simulink model "Stufe5_Laengsdyn3DOF"  (R2026b)
settings: Solver=ode45  StopTime=4.5  MaxStep=0.01  RelTol=1e-6
undefined symbols (not defined in the file or in its folder): PAR_Ach_AbstHi_f64, PAR_Ach_AbstVo_f64, PAR_Ach_BeschlBrems_f64, PAR_Ach_SchwerpHoehe_f64, PAR_Ach_ZeitBrems_f64, PAR_Auf_DaempfHi_f64, PAR_Auf_DaempfVo_f64, PAR_Auf_FederHi_f64, PAR_Auf_FederVo_f64, PAR_Auf_TraeghNick_f64, PAR_Lng_BeschlErde_f64, PAR_Lng_GeschwStart_f64, PAR_Lng_MasseFzg_f64
libraries: simulink x1

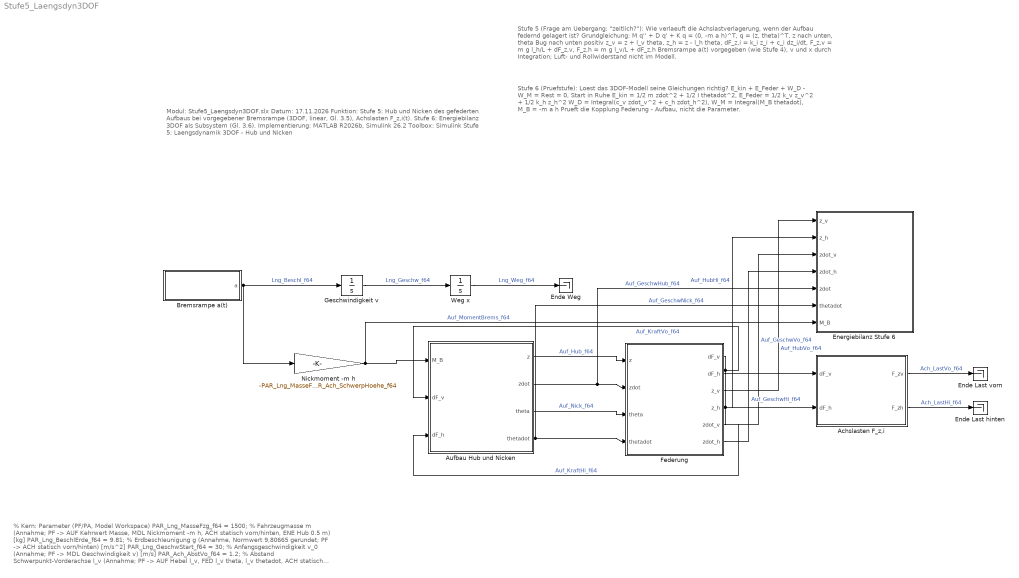
== system Stufe5_Laengsdyn3DOF ==
  note: % Kern: Parameter (PF/PA, Model Workspace)
      | PAR_Lng_MasseFzg_f64 = 1500; % Fahrzeugmasse m (Annahme; PF -> AUF Kehrwert Masse, MDL Nickmoment -m h, ACH statisch vorn/hinten, ENE Hub 0.5 m) [kg]
      | PAR_Lng_BeschlErde_f64 = 9.81; % Erdbeschleunigung g (Annahme, Normwert 9,80665 gerundet; PF -> ACH statisch vorn/hinten) [m/s^2]
      | PAR_Lng_GeschwStart_f64 = 30; % Anfangsgeschwindigkeit v_0 (Annahme; PF -> MDL Geschwindigkeit v) [m/s]
      | PAR_Ach_AbstVo_f64 = 1.2; % Abstand Schwerpunkt-Vorderachse l_v (Annahme; PF -> AUF Hebel l_v, FED l_v theta, l_v thetadot, ACH statisch vorn/hinten) [m]
      | PAR_Ach_AbstHi_f64 = 1.5; % Abstand Schwerpunkt-Hinterachse l_h (Annahme; PF -> AUF Hebel l_h, FED l_h theta, l_h thetadot, ACH statisch vorn/hinten) [m]
      | PAR_Ach_SchwerpHoehe_f64 = 0.55; % Schwerpunkthoehe h (Lit [MW14, Abb. 8.5], Interpretation; PF -> MDL Nickmoment -m h) [m]
      | PAR_Ach_BeschlBrems_f64 = 8; % Betrag der Bremsverzoegerung a_B (Annahme; PA -> BR Rampe, Begrenzung -a_B) [m/s^2]
      | PAR_Ach_ZeitBrems_f64 = 0.3; % Aufbauzeit der Bremsverzoegerung t_r (Annahme; PA -> BR Rampe) [s]
      | PAR_Ach_ZeitStart_f64 = 1; % Beginn der Bremsrampe (Annahme; PA -> BR Rampe) [s]
      | PAR_Auf_FederVo_f64 = 50000; % Federkonstante Vorderachse k_v, beide Raeder (Annahme; PA -> FED Feder k_v, ENE Feder 0.5 k_v) [N/m]
      | PAR_Auf_FederHi_f64 = 45000; % Federkonstante Hinterachse k_h, beide Raeder (Annahme; PA -> FED Feder k_h, ENE Feder 0.5 k_h) [N/m]
      | PAR_Auf_DaempfVo_f64 = 4000; % Daempferkonstante Vorderachse c_v, beide Raeder (Annahme; PA -> FED Daempfer c_v, ENE Daempfer c_v) [N s/m]
      | PAR_Auf_DaempfHi_f64 = 4000; % Daempferkonstante Hinterachse c_h, beide Raeder (Annahme; PA -> FED Daempfer c_h, ENE Daempfer c_h) [N s/m]
      | PAR_Auf_TraeghNick_f64 = 2500; % Nicktraegheitsmoment I um die Querachse (Annahme; PA -> AUF Kehrwert I, ENE Nicken 0.5 I) [kg m^2]
      | % Kern: Signale Stufe 5 (MDL)
      | Lng_Beschl_f64 = '0 -> -8' ; % Beschleunigung a, Bremsrampe, geloggt (MDL; Bremsrampe a(t):1 -> Geschwindigkeit v:1, Nickmoment -m h:1) [m/s^2]
      | Lng_Geschw_f64 = '30 -> 3.2' ; % Geschwindigkeit v, geloggt (MDL; Geschwindigkeit v:1 -> Weg x:1) [m/s]
      | Lng_Weg_f64 = '0 -> 90.08' ; % Weg x, geloggt (MDL; Weg x:1 -> Ende Weg:1) [m]
      | Auf_MomentBrems_f64 = '0 -> 6600' ; % Nickmoment -m a h, geloggt (MDL; Nickmoment -m h:1 -> Aufbau Hub und Nicken:1, Energiebilanz Stufe 6:7) [N m]
      | Auf_Hub_f64 = '0 -> 0.0030 (max 0.0054)' ; % Hub z, nach unten positiv, geloggt (MDL; Aufbau Hub und Nicken:1 -> Federung:1) [m]
      | Auf_GeschwHub_f64 = '0 -> 0 (max 0.0177)' ; % Hubgeschwindigkeit zdot, geloggt (MDL; Aufbau Hub und Nicken:2 -> Federung:2, Energiebilanz Stufe 6:5) [m/s]
      | Auf_Nick_f64 = '0 -> 0.0382 (max 0.0473)' ; % Nickwinkel theta, Bug nach unten positiv, geloggt (MDL; Aufbau Hub und Nicken:3 -> Federung:3) [rad]
      | Auf_GeschwNick_f64 = '0 -> 0 (max 0.154)' ; % Nickgeschwindigkeit thetadot, geloggt (MDL; Aufbau Hub und Nicken:4 -> Federung:4, Energiebilanz Stufe 6:6) [rad/s]
      | Auf_KraftVo_f64 = '0 -> 2444 (max 3261)' ; % Federungskraft vorn dF_z,v = k_v z_v + c_v zdot_v (MDL; Federung:1 -> Aufbau Hub und Nicken:2, Achslasten F_z,i:1) [N]
      | Auf_KraftHi_f64 = '0 -> -2444 (min -3147)' ; % Federungskraft hinten dF_z,h = k_h z_h + c_h zdot_h (MDL; Federung:2 -> Aufbau Hub und Nicken:3, Achslasten F_z,i:2) [N]
      | Ach_LastVo_f64 = '8175 -> 10619 (max 11436)' ; % Achslast vorn F_z,v = m g l_h/L + dF_z,v, geloggt (MDL; Achslasten F_z,i:1 -> Ende Last vorn:1) [N]
      | Ach_LastHi_f64 = '6540 -> 4095 (min 3393)' ; % Achslast hinten F_z,h = m g l_v/L + dF_z,h, geloggt (MDL; Achslasten F_z,i:2 -> Ende Last hinten:1) [N]
  note: Modul: Stufe5_Laengsdyn3DOF.slx
      | Datum: 17.11.2026
      | Funktion: Stufe 5: Hub und Nicken des gefederten Aufbaus bei vorgegebener
      | Bremsrampe (3DOF, linear, Gl. 3.5), Achslasten F_z,i(t).
      | Stufe 6: Energiebilanz 3DOF als Subsystem (Gl. 3.6).
      | Implementierung: MATLAB R2026b, Simulink 26.2
      | Toolbox: Simulink
      |
      | Stufe 5: Laengsdynamik 3DOF - Hub und Nicken
  note: Stufe 5 (Frage am Uebergang: "zeitlich?"): Wie verlaeuft die Achslastverlagerung, wenn der Aufbau federnd gelagert ist?
      | Grundgleichung: M q'' + D q' + K q = (0, -m a h)^T, q = (z, theta)^T, z nach unten, theta Bug nach unten positiv
      | z_v = z + l_v theta, z_h = z - l_h theta, dF_z,i = k_i z_i + c_i dz_i/dt, F_z,v = m g l_h/L + dF_z,v, F_z,h = m g l_v/L + dF_z,h
      | Bremsrampe a(t) vorgegeben (wie Stufe 4), v und x durch Integration; Luft- und Rollwiderstand nicht im Modell.
  note: Stufe 6 (Pruefstufe): Loest das 3DOF-Modell seine Gleichungen richtig?
      | E_kin + E_Feder + W_D - W_M = Rest = 0, Start in Ruhe
      | E_kin = 1/2 m zdot^2 + 1/2 I thetadot^2, E_Feder = 1/2 k_v z_v^2 + 1/2 k_h z_h^2
      | W_D = Integral(c_v zdot_v^2 + c_h zdot_h^2), W_M = Integral(M_B thetadot), M_B = -m a h
      | Prueft die Kopplung Federung - Aufbau, nicht die Parameter.
  Achslasten F_z,i : Subsystem
  Aufbau Hub und Nicken : Subsystem
  Bremsrampe a(t) : Subsystem
  Ende Last hinten : Terminator
  Ende Last vorn : Terminator
  Ende Weg : Terminator
  Energiebilanz Stufe 6 : Subsystem
  Federung : Subsystem
  Geschwindigkeit v : Integrator  InitialCondition=PAR_Lng_GeschwStart_f64
  Nickmoment -m h : Gain  Gain=-PAR_Lng_MasseFzg_f64*PAR_Ach_SchwerpHoehe_f64
  Weg x : Integrator
  wires:
  Bremsrampe a(t)/1(a) -> Geschwindigkeit v/1, Nickmoment -m h/1  "Lng_Beschl_f64"
  Geschwindigkeit v/1 -> Weg x/1  "Lng_Geschw_f64"
  Weg x/1 -> Ende Weg/1  "Lng_Weg_f64"
  Nickmoment -m h/1 -> Aufbau Hub und Nicken/1(M_B), Energiebilanz Stufe 6/7(M_B)  "Auf_MomentBrems_f64"
  Aufbau Hub und Nicken/1(z) -> Federung/1(z)  "Auf_Hub_f64"
  Aufbau Hub und Nicken/2(zdot) -> Federung/2(zdot), Energiebilanz Stufe 6/5(zdot)  "Auf_GeschwHub_f64"
  Aufbau Hub und Nicken/3(theta) -> Federung/3(theta)  "Auf_Nick_f64"
  Aufbau Hub und Nicken/4(thetadot) -> Federung/4(thetadot), Energiebilanz Stufe 6/6(thetadot)  "Auf_GeschwNick_f64"
  Federung/1(dF_v) -> Aufbau Hub und Nicken/2(dF_v), Achslasten F_z,i/1(dF_v)  "Auf_KraftVo_f64"
  Federung/2(dF_h) -> Aufbau Hub und Nicken/3(dF_h), Achslasten F_z,i/2(dF_h)  "Auf_KraftHi_f64"
  Achslasten F_z,i/1(F_zv) -> Ende Last vorn/1  "Ach_LastVo_f64"
  Achslasten F_z,i/2(F_zh) -> Ende Last hinten/1  "Ach_LastHi_f64"
  Federung/3(z_v) -> Energiebilanz Stufe 6/1(z_v)  "Auf_HubVo_f64"
  Federung/4(z_h) -> Energiebilanz Stufe 6/2(z_h)  "Auf_HubHi_f64"
  Federung/5(zdot_v) -> Energiebilanz Stufe 6/3(zdot_v)  "Auf_GeschwVo_f64"
  Federung/6(zdot_h) -> Energiebilanz Stufe 6/4(zdot_h)  "Auf_GeschwHi_f64"

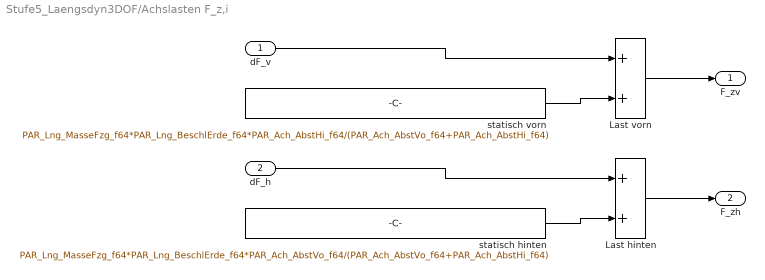
== system Stufe5_Laengsdyn3DOF/Achslasten F_z,i ==
  dF_v : Inport
  dF_h : Inport  Port=2
  Last hinten : Sum
  Last vorn : Sum
  statisch hinten : Constant  Value=PAR_Lng_MasseFzg_f64*PAR_Lng_BeschlErde_f64*PAR_Ach_AbstVo_f64/(PAR_Ach_AbstVo_f64+PAR_Ach_AbstHi_f64)
  statisch vorn : Constant  Value=PAR_Lng_MasseFzg_f64*PAR_Lng_BeschlErde_f64*PAR_Ach_AbstHi_f64/(PAR_Ach_AbstVo_f64+PAR_Ach_AbstHi_f64)
  F_zv : Outport
  F_zh : Outport  Port=2
  wires:
  dF_v/1 -> Last vorn/1
  statisch vorn/1 -> Last vorn/2
  dF_h/1 -> Last hinten/1
  statisch hinten/1 -> Last hinten/2
  Last vorn/1 -> F_zv/1
  Last hinten/1 -> F_zh/1

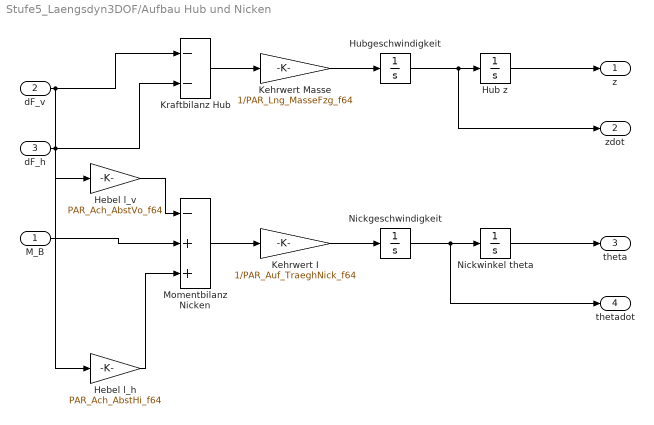
== system Stufe5_Laengsdyn3DOF/Aufbau Hub und Nicken ==
  M_B : Inport
  dF_v : Inport  Port=2
  dF_h : Inport  Port=3
  Hebel l_h : Gain  Gain=PAR_Ach_AbstHi_f64
  Hebel l_v : Gain  Gain=PAR_Ach_AbstVo_f64
  Hub z : Integrator
  Hubgeschwindigkeit : Integrator
  Kehrwert I : Gain  Gain=1/PAR_Auf_TraeghNick_f64
  Kehrwert Masse : Gain  Gain=1/PAR_Lng_MasseFzg_f64
  Kraftbilanz Hub : Sum  Inputs=|--
  Momentbilanz Nicken : Sum  Inputs=-++
  Nickgeschwindigkeit : Integrator
  Nickwinkel theta : Integrator
  z : Outport
  zdot : Outport  Port=2
  theta : Outport  Port=3
  thetadot : Outport  Port=4
  wires:
  dF_v/1 -> Kraftbilanz Hub/1, Hebel l_v/1
  dF_h/1 -> Kraftbilanz Hub/2, Hebel l_h/1
  Kraftbilanz Hub/1 -> Kehrwert Masse/1
  Kehrwert Masse/1 -> Hubgeschwindigkeit/1
  Hubgeschwindigkeit/1 -> Hub z/1, zdot/1
  Hub z/1 -> z/1
  Hebel l_v/1 -> Momentbilanz Nicken/1
  M_B/1 -> Momentbilanz Nicken/2
  Hebel l_h/1 -> Momentbilanz Nicken/3
  Momentbilanz Nicken/1 -> Kehrwert I/1
  Kehrwert I/1 -> Nickgeschwindigkeit/1
  Nickgeschwindigkeit/1 -> Nickwinkel theta/1, thetadot/1
  Nickwinkel theta/1 -> theta/1

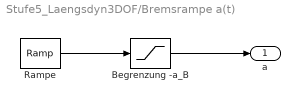
== system Stufe5_Laengsdyn3DOF/Bremsrampe a(t) ==
  Begrenzung -a_B : Saturate  UpperLimit=0  LowerLimit=-PAR_Ach_BeschlBrems_f64
  Rampe : simulink/Sources/Ramp  slope=-PAR_Ach_BeschlBrems_f64/PAR_Ach_ZeitBrems_f64  start=PAR_Ach_ZeitStart_f64  InitialOutput=0
  a : Outport
  wires:
  Rampe/1 -> Begrenzung -a_B/1
  Begrenzung -a_B/1 -> a/1

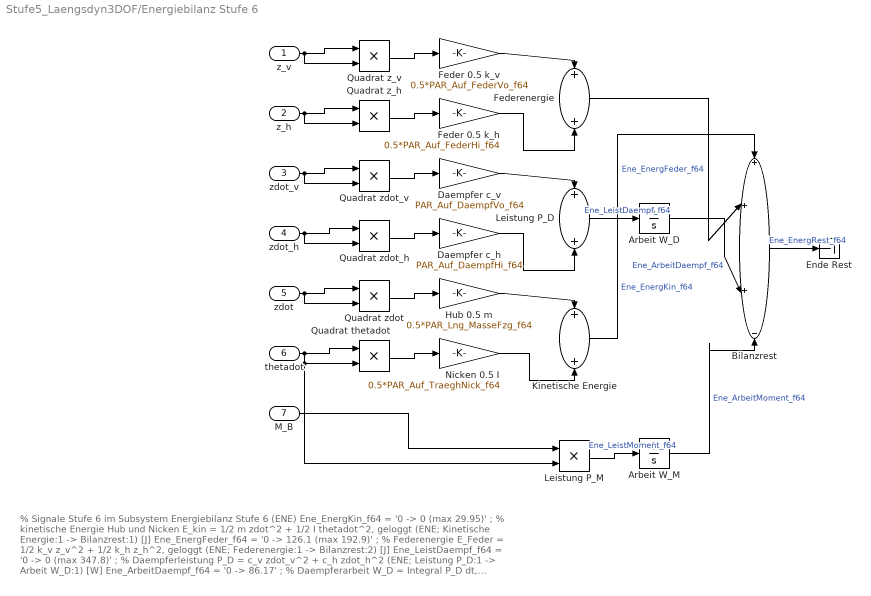
== system Stufe5_Laengsdyn3DOF/Energiebilanz Stufe 6 ==
  note: % Signale Stufe 6 im Subsystem Energiebilanz Stufe 6 (ENE)
      | Ene_EnergKin_f64 = '0 -> 0 (max 29.95)' ; % kinetische Energie Hub und Nicken E_kin = 1/2 m zdot^2 + 1/2 I thetadot^2, geloggt (ENE; Kinetische Energie:1 -> Bilanzrest:1) [J]
      | Ene_EnergFeder_f64 = '0 -> 126.1 (max 192.9)' ; % Federenergie E_Feder = 1/2 k_v z_v^2 + 1/2 k_h z_h^2, geloggt (ENE; Federenergie:1 -> Bilanzrest:2) [J]
      | Ene_LeistDaempf_f64 = '0 -> 0 (max 347.8)' ; % Daempferleistung P_D = c_v zdot_v^2 + c_h zdot_h^2 (ENE; Leistung P_D:1 -> Arbeit W_D:1) [W]
      | Ene_ArbeitDaempf_f64 = '0 -> 86.17' ; % Daempferarbeit W_D = Integral P_D dt, geloggt (ENE; Arbeit W_D:1 -> Bilanzrest:3) [J]
      | Ene_LeistMoment_f64 = '0 -> 0 (max 1019, min -312)' ; % Leistung des Nickmoments P_M = M_B thetadot (ENE; Leistung P_M:1 -> Arbeit W_M:1) [W]
      | Ene_ArbeitMoment_f64 = '0 -> 212.3 (max 271.9)' ; % Arbeit des Nickmoments W_M = Integral P_M dt, geloggt (ENE; Arbeit W_M:1 -> Bilanzrest:4) [J]
      | Ene_EnergRest_f64 = '0 -> -2.9e-07' ; % Bilanzrest E_kin + E_Feder + W_D - W_M, geloggt, Toleranz 3.9e-04 J (ENE; Bilanzrest:1 -> Ende Rest:1) [J]
  z_v : Inport
  z_h : Inport  Port=2
  zdot_v : Inport  Port=3
  zdot_h : Inport  Port=4
  zdot : Inport  Port=5
  thetadot : Inport  Port=6
  M_B : Inport  Port=7
  Arbeit W_D : Integrator
  Arbeit W_M : Integrator
  Bilanzrest : Sum  Inputs=+++-
  Daempfer c_h : Gain  Gain=PAR_Auf_DaempfHi_f64
  Daempfer c_v : Gain  Gain=PAR_Auf_DaempfVo_f64
  Ende Rest : Terminator
  Feder 0.5 k_h : Gain  Gain=0.5*PAR_Auf_FederHi_f64
  Feder 0.5 k_v : Gain  Gain=0.5*PAR_Auf_FederVo_f64
  Federenergie : Sum
  Hub 0.5 m : Gain  Gain=0.5*PAR_Lng_MasseFzg_f64
  Kinetische Energie : Sum
  Leistung P_D : Sum
  Leistung P_M : Product
  Nicken 0.5 I : Gain  Gain=0.5*PAR_Auf_TraeghNick_f64
  Quadrat thetadot : Product
  Quadrat z_h : Product
  Quadrat z_v : Product
  Quadrat zdot : Product
  Quadrat zdot_h : Product
  Quadrat zdot_v : Product
  wires:
  z_v/1 -> Quadrat z_v/1, Quadrat z_v/2
  Quadrat z_v/1 -> Feder 0.5 k_v/1
  z_h/1 -> Quadrat z_h/1, Quadrat z_h/2
  Quadrat z_h/1 -> Feder 0.5 k_h/1
  zdot_v/1 -> Quadrat zdot_v/1, Quadrat zdot_v/2
  Quadrat zdot_v/1 -> Daempfer c_v/1
  zdot_h/1 -> Quadrat zdot_h/1, Quadrat zdot_h/2
  Quadrat zdot_h/1 -> Daempfer c_h/1
  zdot/1 -> Quadrat zdot/1, Quadrat zdot/2
  Quadrat zdot/1 -> Hub 0.5 m/1
  thetadot/1 -> Quadrat thetadot/2, Leistung P_M/2, Quadrat thetadot/1
  Quadrat thetadot/1 -> Nicken 0.5 I/1
  Feder 0.5 k_v/1 -> Federenergie/1
  Feder 0.5 k_h/1 -> Federenergie/2
  Daempfer c_v/1 -> Leistung P_D/1
  Daempfer c_h/1 -> Leistung P_D/2
  Hub 0.5 m/1 -> Kinetische Energie/1
  M_B/1 -> Leistung P_M/1
  Leistung P_D/1 -> Arbeit W_D/1  "Ene_LeistDaempf_f64"
  Leistung P_M/1 -> Arbeit W_M/1  "Ene_LeistMoment_f64"
  Kinetische Energie/1 -> Bilanzrest/1  "Ene_EnergKin_f64"
  Federenergie/1 -> Bilanzrest/2  "Ene_EnergFeder_f64"
  Arbeit W_D/1 -> Bilanzrest/3  "Ene_ArbeitDaempf_f64"
  Bilanzrest/1 -> Ende Rest/1  "Ene_EnergRest_f64"
  Nicken 0.5 I/1 -> Kinetische Energie/2
  Arbeit W_M/1 -> Bilanzrest/4  "Ene_ArbeitMoment_f64"

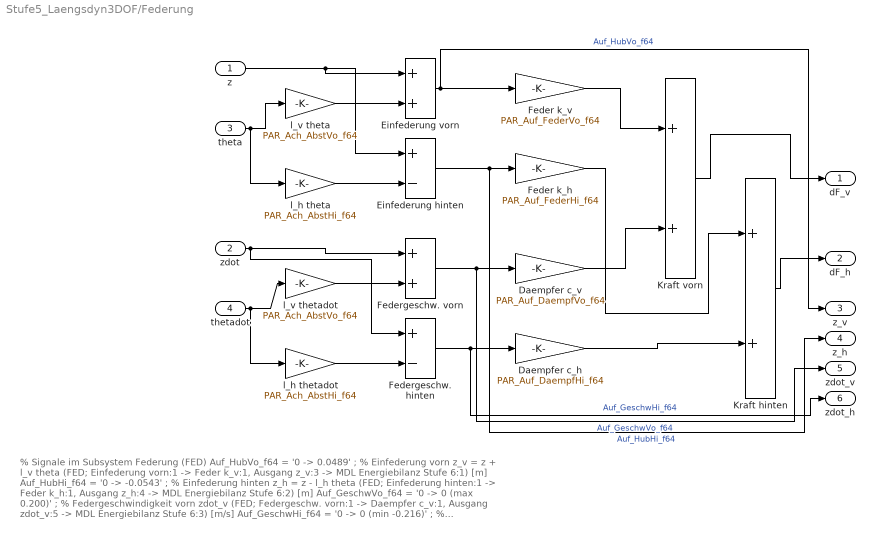
== system Stufe5_Laengsdyn3DOF/Federung ==
  note: % Signale im Subsystem Federung (FED)
      | Auf_HubVo_f64 = '0 -> 0.0489' ; % Einfederung vorn z_v = z + l_v theta (FED; Einfederung vorn:1 -> Feder k_v:1, Ausgang z_v:3 -> MDL Energiebilanz Stufe 6:1) [m]
      | Auf_HubHi_f64 = '0 -> -0.0543' ; % Einfederung hinten z_h = z - l_h theta (FED; Einfederung hinten:1 -> Feder k_h:1, Ausgang z_h:4 -> MDL Energiebilanz Stufe 6:2) [m]
      | Auf_GeschwVo_f64 = '0 -> 0 (max 0.200)' ; % Federgeschwindigkeit vorn zdot_v (FED; Federgeschw. vorn:1 -> Daempfer c_v:1, Ausgang zdot_v:5 -> MDL Energiebilanz Stufe 6:3) [m/s]
      | Auf_GeschwHi_f64 = '0 -> 0 (min -0.216)' ; % Federgeschwindigkeit hinten zdot_h (FED; Federgeschw. hinten:1 -> Daempfer c_h:1, Ausgang zdot_h:6 -> MDL Energiebilanz Stufe 6:4) [m/s]
  z : Inport
  zdot : Inport  Port=2
  theta : Inport  Port=3
  thetadot : Inport  Port=4
  Daempfer c_h : Gain  Gain=PAR_Auf_DaempfHi_f64
  Daempfer c_v : Gain  Gain=PAR_Auf_DaempfVo_f64
  Einfederung hinten : Sum  Inputs=+-
  Einfederung vorn : Sum
  Feder k_h : Gain  Gain=PAR_Auf_FederHi_f64
  Feder k_v : Gain  Gain=PAR_Auf_FederVo_f64
  Federgeschw. hinten : Sum  Inputs=+-
  Federgeschw. vorn : Sum
  Kraft hinten : Sum
  Kraft vorn : Sum
  l_h theta : Gain  Gain=PAR_Ach_AbstHi_f64
  l_h thetadot : Gain  Gain=PAR_Ach_AbstHi_f64
  l_v theta : Gain  Gain=PAR_Ach_AbstVo_f64
  l_v thetadot : Gain  Gain=PAR_Ach_AbstVo_f64
  dF_v : Outport
  dF_h : Outport  Port=2
  z_v : Outport  Port=3
  z_h : Outport  Port=4
  zdot_v : Outport  Port=5
  zdot_h : Outport  Port=6
  wires:
  theta/1 -> l_v theta/1, l_h theta/1
  thetadot/1 -> l_v thetadot/1, l_h thetadot/1
  z/1 -> Einfederung vorn/1, Einfederung hinten/1
  l_v theta/1 -> Einfederung vorn/2
  l_h theta/1 -> Einfederung hinten/2
  zdot/1 -> Federgeschw. vorn/1, Federgeschw. hinten/1
  l_v thetadot/1 -> Federgeschw. vorn/2
  l_h thetadot/1 -> Federgeschw. hinten/2
  Einfederung vorn/1 -> Feder k_v/1, z_v/1  "Auf_HubVo_f64"
  Einfederung hinten/1 -> Feder k_h/1, z_h/1  "Auf_HubHi_f64"
  Federgeschw. vorn/1 -> Daempfer c_v/1, zdot_v/1  "Auf_GeschwVo_f64"
  Federgeschw. hinten/1 -> Daempfer c_h/1, zdot_h/1  "Auf_GeschwHi_f64"
  Feder k_v/1 -> Kraft vorn/1
  Daempfer c_v/1 -> Kraft vorn/2
  Feder k_h/1 -> Kraft hinten/1
  Daempfer c_h/1 -> Kraft hinten/2
  Kraft vorn/1 -> dF_v/1
  Kraft hinten/1 -> dF_h/1
